simulink model "BLDC"  (R2021a)
settings: Solver=VariableStepAuto  StartTime=0.0  StopTime=2  MaxStep=1e-4  RelTol=1e-3
undefined symbols (not defined in the file or in its folder): B, J, Ke, Ls, p, pm, Rs
libraries: spsVoltageMeasurementLib x2, spsDCVoltageSourceLib x1, spsUniversalBridgeLib x1, spspowerguiLib x1
settings Model: Creator=musta  LastModifiedBy=musta

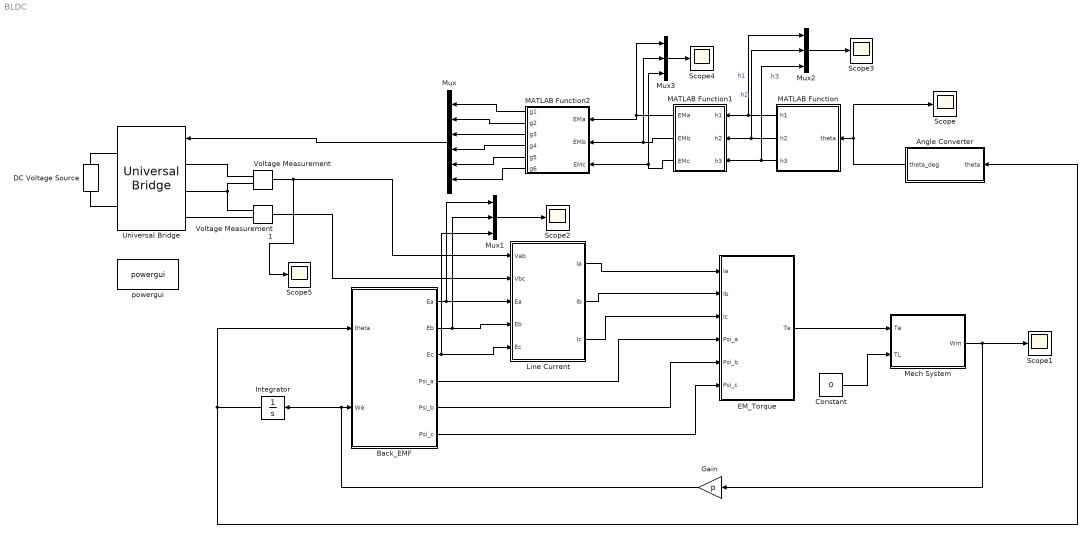
== system BLDC ==
  note: h3
  Angle Converter : Subsystem
  Back_EMF : Subsystem
  Constant : Constant  Value=0
  DC Voltage Source : spsDCVoltageSourceLib/DC Voltage Source  Amplitude=240  Measurements=None
  EM_Torque : Subsystem
  Gain : Gain  Gain=p
  Integrator : Integrator
  Line Current : Subsystem
  MATLAB Function : MATLAB Function  TreatAsAtomicUnit=on
  MATLAB Function1 : MATLAB Function  TreatAsAtomicUnit=on
  MATLAB Function2 : MATLAB Function  TreatAsAtomicUnit=on
  Mech System : Subsystem
  Mux : Mux  Inputs=6
  Mux1 : Mux  Inputs=3
  Mux2 : Mux  Inputs=3
  Mux3 : Mux  Inputs=3
  Scope{,1..5} (6 alike) : Scope
  Universal Bridge : spsUniversalBridgeLib/Universal Bridge  Arms=3  SnubberResistance=1e5  SnubberCapacitance=inf  Device=IGBT / Diodes  Ron=1e-3  Lon=0  ForwardVoltages="[  0  0  ]"  ForwardVoltage=0  GTOparameters=[ 10e-6 , 20e-6 ]  IGBTparameters=[ 1e-6 , 2e-6 ]  Measurements=None  Measurements_2=None  converterType=Rectifier
  Voltage Measurement : spsVoltageMeasurementLib/Voltage Measurement  PhasorSimulation=off  OutputType=Complex  PSBequivalent=0
  Voltage Measurement1 : spsVoltageMeasurementLib/Voltage Measurement  PhasorSimulation=off  OutputType=Complex  PSBequivalent=0
  powergui : spspowerguiLib/powergui  Priority=1  SimulationMode=Continuous  SampleTime=50e-6  frequency=60  Iterations=50  frequencyindice=0  Pbase=100e6  ErrMax=1e-4  UnitsV=kV  UnitsW=MW  buscounter=0  FunctionMessages=off  echomessages=off  EnableUseOfTLC=off  CurrentSourceSwitches=off  DisableSnubberDevices=off  DisableRonSwitches=off  DisableVfSwitches=off  DisplayEquations=off  AutomaticDiscreteSolvers=off  SolverType=Tustin/Backward Euler (TBE)  Interpol=off  ExternalGateDelay=off  methode=off  Ts=100  x0status=blocks  SPID=on  SwTol=0  HookPort=off  NonlinearTolerance=1e-4  nMaxIteration=100  ContinueOnMaxIteration=off  RestoreLinks=warning  ResistiveCurrentMeasurement=off  Frange=[0:2:500]  Ylog=off  Xlog=on  ShowGrid=off  save=off  variable=ZData  structure=0  ZoomFFT=off  StartTime=0.0  cycles=1  DisplayStyle=1  fundamental=60  FreqAxis=off  MaxFrequency=1000  frequencyindicesteady=1  RmsSteady=1  display=off
  wires:
  Back_EMF/1(Ea) -> Mux1/1, Line Current/3(Ea)
  Back_EMF/2(Eb) -> Mux1/2, Line Current/4(Eb)
  Back_EMF/3(Ec) -> Line Current/5(Ec), Mux1/3
  Line Current/1(Ia) -> EM_Torque/1(Ia)
  Line Current/2(Ib) -> EM_Torque/2(Ib)
  Line Current/3(Ic) -> EM_Torque/3(Ic)
  Back_EMF/4(Psi_a) -> EM_Torque/4(Psi_a)
  Back_EMF/5(Psi_b) -> EM_Torque/5(Psi_b)
  Back_EMF/6(Psi_c) -> EM_Torque/6(Psi_c)
  EM_Torque/1(Te) -> Mech System/1(Te)
  Integrator/1 -> Angle Converter/1(theta), Back_EMF/1(theta)
  Mech System/1(Wm) -> Gain/1, Scope1/1
  Gain/1 -> Back_EMF/2(We), Integrator/1
  Constant/1 -> Mech System/2(TL)
  Voltage Measurement/1 -> Scope5/1, Line Current/1(Vab)
  Voltage Measurement1/1 -> Line Current/2(Vbc)
  Angle Converter/1(theta_deg) -> Scope/1, MATLAB Function/1(theta)
  MATLAB Function/1(h1) -> Mux2/1, MATLAB Function1/1(h1)  "h1"
  MATLAB Function/2(h2) -> Mux2/2, MATLAB Function1/2(h2)  "h2"
  MATLAB Function/3(h3) -> MATLAB Function1/3(h3), Mux2/3
  MATLAB Function1/1(EMa) -> Mux3/1, MATLAB Function2/1(EMa)
  MATLAB Function1/2(EMb) -> Mux3/2, MATLAB Function2/2(EMb)
  MATLAB Function1/3(EMc) -> Mux3/3, MATLAB Function2/3(EMc)
  Mux/1 -> Universal Bridge/1
  MATLAB Function2/1(g1) -> Mux/1
  MATLAB Function2/2(g2) -> Mux/2
  MATLAB Function2/3(g3) -> Mux/3
  MATLAB Function2/4(g4) -> Mux/4
  MATLAB Function2/5(g5) -> Mux/5
  MATLAB Function2/6(g6) -> Mux/6
  Mux1/1 -> Scope2/1
  Mux2/1 -> Scope3/1
  Mux3/1 -> Scope4/1
  connections:
  DC Voltage Source/RConn1 -- Universal Bridge/RConn1
  DC Voltage Source/LConn1 -- Universal Bridge/RConn2
  Universal Bridge/LConn1 -- Voltage Measurement/LConn1
  Universal Bridge/LConn3 -- Voltage Measurement1/LConn2
  Universal Bridge/LConn2 -- Voltage Measurement1/LConn1 -- Voltage Measurement/LConn2

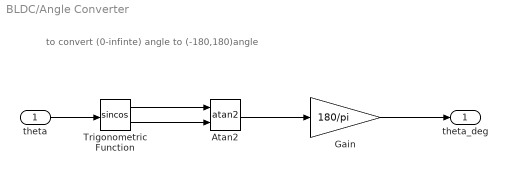
== system BLDC/Angle Converter ==
  note: to convert (0-infinte) angle to (-180,180)angle
  theta : Inport
  Atan2 : Trigonometry  Operator=atan2
  Gain : Gain  Gain=180/pi
  Trigonometric Function : Trigonometry  Operator=sincos
  theta_deg : Outport
  wires:
  Atan2/1 -> Gain/1
  Gain/1 -> theta_deg/1
  theta/1 -> Trigonometric Function/1
  Trigonometric Function/1 -> Atan2/1
  Trigonometric Function/2 -> Atan2/2

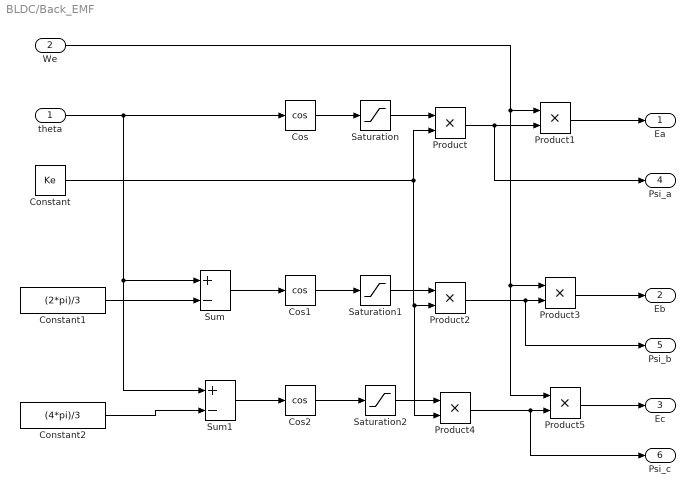
== system BLDC/Back_EMF ==
  theta : Inport
  We : Inport  Port=2
  Constant : Constant  Value=Ke
  Constant1 : Constant  Value=(2*pi)/3
  Constant2 : Constant  Value=(4*pi)/3
  Cos : Trigonometry  Operator=cos
  Cos1 : Trigonometry  Operator=cos
  Cos2 : Trigonometry  Operator=cos
  Product{,1..5} (6 alike) : Product
  Saturation : Saturate  UpperLimit=0.45  LowerLimit=-0.45
  Saturation1 : Saturate  UpperLimit=0.45  LowerLimit=-0.45
  Saturation2 : Saturate  UpperLimit=0.45  LowerLimit=-0.45
  Sum : Sum  Inputs=+-
  Sum1 : Sum  Inputs=+-
  Ea : Outport
  Eb : Outport  Port=2
  Ec : Outport  Port=3
  Psi_a : Outport  Port=4
  Psi_b : Outport  Port=5
  Psi_c : Outport  Port=6
  wires:
  theta/1 -> Cos/1, Sum1/1, Sum/1
  Cos/1 -> Saturation/1
  Saturation/1 -> Product/1
  Product/1 -> Psi_a/1, Product1/2
  We/1 -> Product5/1, Product3/1, Product1/1
  Product1/1 -> Ea/1
  Constant/1 -> Product4/2, Product2/2, Product/2
  Constant1/1 -> Sum/2
  Sum/1 -> Cos1/1
  Cos1/1 -> Saturation1/1
  Saturation1/1 -> Product2/1
  Product2/1 -> Psi_b/1, Product3/2
  Product3/1 -> Eb/1
  Product4/1 -> Psi_c/1, Product5/2
  Saturation2/1 -> Product4/1
  Cos2/1 -> Saturation2/1
  Sum1/1 -> Cos2/1
  Constant2/1 -> Sum1/2
  Product5/1 -> Ec/1

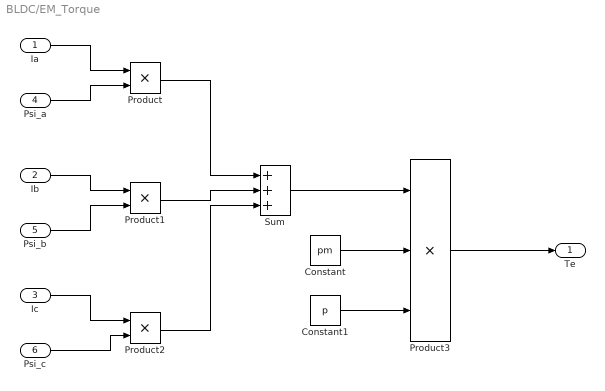
== system BLDC/EM_Torque ==
  Ia : Inport
  Ib : Inport  Port=2
  Ic : Inport  Port=3
  Psi_a : Inport  Port=4
  Psi_b : Inport  Port=5
  Psi_c : Inport  Port=6
  Constant : Constant  Value=pm
  Constant1 : Constant  Value=p
  Product : Product
  Product1 : Product
  Product2 : Product
  Product3 : Product  Inputs=3
  Sum : Sum  Inputs=+++
  Te : Outport
  wires:
  Ia/1 -> Product/1
  Psi_a/1 -> Product/2
  Ib/1 -> Product1/1
  Psi_b/1 -> Product1/2
  Ic/1 -> Product2/1
  Psi_c/1 -> Product2/2
  Product/1 -> Sum/1
  Product1/1 -> Sum/2
  Product2/1 -> Sum/3
  Sum/1 -> Product3/1
  Constant/1 -> Product3/2
  Constant1/1 -> Product3/3
  Product3/1 -> Te/1

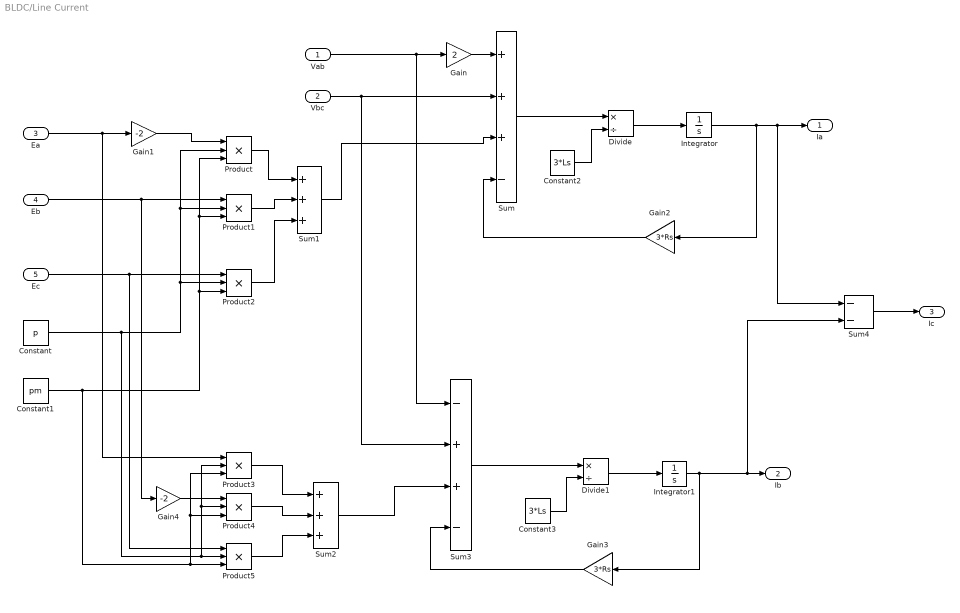
== system BLDC/Line Current ==
  Vab : Inport
  Vbc : Inport  Port=2
  Ea : Inport  Port=3
  Eb : Inport  Port=4
  Ec : Inport  Port=5
  Constant : Constant  Value=p
  Constant1 : Constant  Value=pm
  Constant2 : Constant  Value=3*Ls
  Constant3 : Constant  Value=3*Ls
  Divide : Product  Inputs=*/
  Divide1 : Product  Inputs=*/
  Gain : Gain  Gain=2
  Gain1 : Gain  Gain=-2
  Gain2 : Gain  Gain=3*Rs
  Gain3 : Gain  Gain=3*Rs
  Gain4 : Gain  Gain=-2
  Integrator : Integrator
  Integrator1 : Integrator
  Product{,1..5} (6 alike) : Product  Inputs=3
  Sum : Sum  Inputs=+++-
  Sum1 : Sum  Inputs=+++
  Sum2 : Sum  Inputs=+++
  Sum3 : Sum  Inputs=-++-
  Sum4 : Sum  Inputs=--
  Ia : Outport
  Ib : Outport  Port=2
  Ic : Outport  Port=3
  wires:
  Vab/1 -> Sum3/1, Gain/1
  Gain/1 -> Sum/1
  Vbc/1 -> Sum3/2, Sum/2
  Ea/1 -> Product3/1, Gain1/1
  Gain1/1 -> Product/1
  Eb/1 -> Gain4/1, Product1/1
  Ec/1 -> Product5/1, Product2/1
  Constant/1 -> Product3/2, Product4/2, Product5/2, Product1/2, Product/2, Product2/2
  Constant1/1 -> Product3/3, Product4/3, Product5/3, Product1/3, Product/3, Product2/3
  Product/1 -> Sum1/1
  Product1/1 -> Sum1/2
  Product2/1 -> Sum1/3
  Sum1/1 -> Sum/3
  Sum/1 -> Divide/1
  Constant2/1 -> Divide/2
  Divide/1 -> Integrator/1
  Integrator/1 -> Gain2/1, Sum4/1, Ia/1
  Gain2/1 -> Sum/4
  Product3/1 -> Sum2/1
  Product4/1 -> Sum2/2
  Product5/1 -> Sum2/3
  Sum2/1 -> Sum3/3
  Divide1/1 -> Integrator1/1
  Constant3/1 -> Divide1/2
  Sum3/1 -> Divide1/1
  Integrator1/1 -> Gain3/1, Sum4/2, Ib/1
  Gain3/1 -> Sum3/4
  Sum4/1 -> Ic/1
  Gain4/1 -> Product4/1

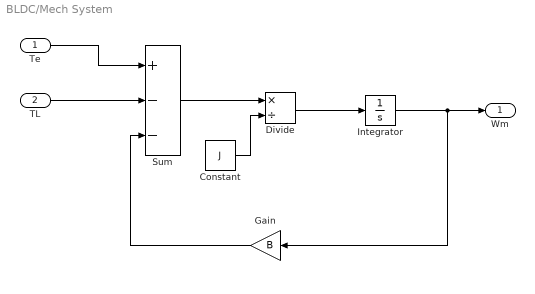
== system BLDC/Mech System ==
  Te : Inport
  TL : Inport  Port=2
  Constant : Constant  Value=J
  Divide : Product  Inputs=*/
  Gain : Gain  Gain=B
  Integrator : Integrator
  Sum : Sum  Inputs=+--
  Wm : Outport
  wires:
  Te/1 -> Sum/1
  TL/1 -> Sum/2
  Sum/1 -> Divide/1
  Constant/1 -> Divide/2
  Divide/1 -> Integrator/1
  Integrator/1 -> Gain/1, Wm/1
  Gain/1 -> Sum/3

== matlab function BLDC/MATLAB Function1 ==
  data: h1 input; EMa output; h2 input; h3 input; EMb output; EMc output
function [EMa, EMb, EMc] = fcn(h1, h2, h3)

if h1==0 && h2==0 && h3==1
    EMa = -1; EMb = 0; EMc = 1;
elseif h1==1 && h2==0 && h3==1
    EMa = 0; EMb = -1; EMc = 1;
elseif h1==1 && h2==0 && h3==0
    EMa = 1; EMb = -1; EMc = 0;
elseif h1==1 && h2==1 && h3==0
    EMa = 1; EMb = 0; EMc = -1;
elseif h1==0 && h2==1 && h3==0
    EMa = 0; EMb = 1; EMc = -1;
elseif h1==0 && h2==1 && h3==1
    EMa = -1; EMb = 1; EMc = 0;
else
    EMa = 0; EMb = 0; EMc = 0;
end

end

== matlab function BLDC/MATLAB Function ==
  data: theta input; h1 output; h2 output; h3 output
function [h1, h2, h3] = fcn(theta)
    
    if theta >= -180 && theta < -120
        h1 = 0; h2 = 0; h3 = 1;
    elseif theta >= -120 && theta < -60
        h1 = 1; h2 = 0; h3 = 1;
    elseif theta >= -60 && theta < 0
        h1 = 1; h2 = 0; h3 = 0;
    elseif theta >= 0 && theta < 60
        h1 = 1; h2 = 1; h3 = 0;
    elseif theta >= 60 && theta < 120
        h1 = 0; h2 = 1; h3 = 0;
    elseif theta >= 120 && theta <= 180
        h1 = 0; h2 = 1; h3 = 1;
    else
        h1 = 0; h2 = 0; h3 = 0;  
    end
    
end

== matlab function BLDC/MATLAB Function2 ==
  data: EMa input; g1 output; EMb input; EMc input; g2 output; g3 output; g4 output; g5 output; g6 output
function [g1, g2, g3, g4, g5, g6] = fcn(EMa, EMb, EMc)

if EMa > 0
    g1 = 1;
else
    g1 = 0;
end

if EMa < 0
    g2 = 1;
else
    g2 = 0;
end

if EMb > 0
    g3 = 1;
else
    g3 = 0;
end

if EMb < 0
    g4 = 1;
else
    g4 = 0;
end

if EMc > 0
    g5 = 1;
else
    g5 = 0;
end

if EMc < 0
    g6 = 1;
else
    g6 = 0;
end

end
